simulink model "ride_demo_halfcar"  (R2025b)
settings: Solver=ode4  StartTime=0.0  StopTime=numel(ride_speeds) * ride_dt  FixedStep=ride_dt_sim  RelTol=1e-3
InitFcn:
  | if isempty(which('ride.run'))
  |     run(fullfile(fileparts(get_param(bdroot, 'FileName')), '..', 'setup.m'));
  | end
  | if ~exist('ride_road', 'var') || ~exist('ride_speeds', 'var')
  |     ride_demo_run = ride.run(ride.config('model', 'halfcar'));
  |     ride_road = ride_demo_run.road;
  |     ride_speeds = ride_demo_run.speeds;
  |     ride_dt = ride_demo_run.P.DT;
  |     ride_dt_sim = ride_demo_run.P.DT_SIM;
  |     clear ride_demo_run
  | end
libraries: ride_lib x4
settings Model: Creator=mohammedazab  LastModifiedBy=mohammedazab
settings DataIOCC: SaveOutput=off  SaveTime=off

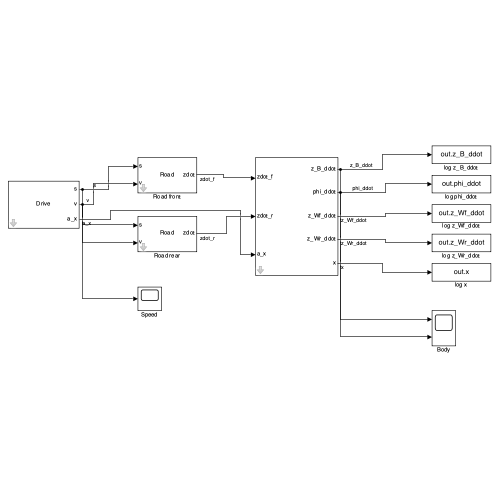
[thumbnail: Simulink's stored preview of the top-level diagram]
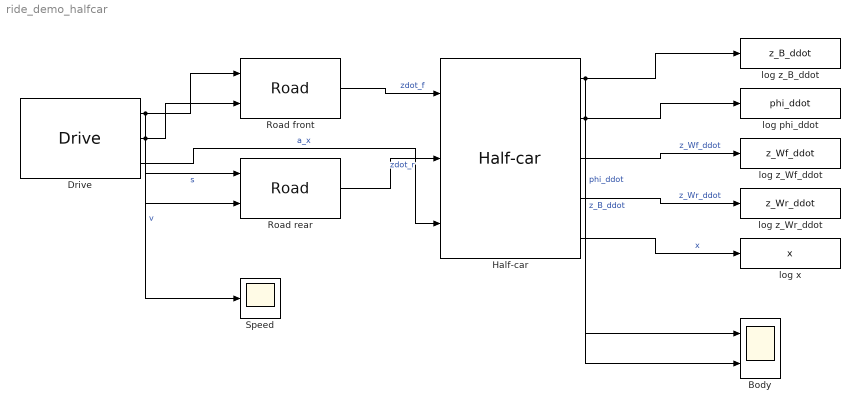
== system ride_demo_halfcar ==
  Body : Scope  NumInputPorts=2
  Drive : ride_lib/Drive  speeds=ride_speeds  dt=ride_dt
  Half-car : ride_lib/Half-car  m_B=803  I_B=1430  l_f=1.206  l_r=1.6639999999999999  h_T=0.59999999999999998  h_B=0.222  front_m_W=50.399999999999999  front_k_T=262200  front_c_T=500  front_k_S=29589.900000000001  front_dz_S_stat=0.16361320259798129  front_dz_cmp=0.02  front_dz_rbd=0.080000000000000002  front_f1_cmp=0.33333333329999998  front_f2_cmp=4  front_f1_rbd=1  front_f2_rbd=8  front_F_max=100000  front_D=564.80000000000007  front_A=0.5  front_v_d=0.20000000000000001  front_v_z=0.20000000000000001  rear_m_W=50.399999999999999  rear_k_T=262200  rear_c_T=500  rear_k_S=21444.860000000001  rear_dz_S_stat=0.16361857789913259  rear_dz_cmp=0.02  rear_dz_rbd=0.080000000000000002  rear_f1_cmp=0.33333333329999998  rear_f2_cmp=4  rear_f1_rbd=1  rear_f2_rbd=8  rear_F_max=100000  rear_D=562.39999999999998  rear_A=0.5  rear_v_d=0.20000000000000001  rear_v_z=0.20000000000000001
  Road front : ride_lib/Road  road=ride_road  lag_m=0
  Road rear : ride_lib/Road  road=ride_road  lag_m=2.8700000000000001
  Speed : Scope
  log phi_ddot : ToWorkspace  VariableName=phi_ddot  SampleTime=ride_dt
  log x : ToWorkspace  VariableName=x  SampleTime=ride_dt
  log z_B_ddot : ToWorkspace  VariableName=z_B_ddot  SampleTime=ride_dt
  log z_Wf_ddot : ToWorkspace  VariableName=z_Wf_ddot  SampleTime=ride_dt
  log z_Wr_ddot : ToWorkspace  VariableName=z_Wr_ddot  SampleTime=ride_dt
  wires:
  Drive/1 -> Road front/1, Road rear/1  "s"
  Drive/2 -> Road front/2, Road rear/2, Speed/1  "v"
  Road front/1 -> Half-car/1  "zdot_f"
  Road rear/1 -> Half-car/2  "zdot_r"
  Drive/3 -> Half-car/3  "a_x"
  Half-car/1 -> log z_B_ddot/1, Body/1  "z_B_ddot"
  Half-car/2 -> log phi_ddot/1, Body/2  "phi_ddot"
  Half-car/3 -> log z_Wf_ddot/1  "z_Wf_ddot"
  Half-car/4 -> log z_Wr_ddot/1  "z_Wr_ddot"
  Half-car/5 -> log x/1  "x"
